simulink model "auv_v3_closed_loop"  (R2024b)
settings: Solver=ode4  StartTime=0.0  StopTime=200  FixedStep=0.02  RelTol=1e-3
model workspace (MAT data in the model file):
  CaseIndex = 1
  ControllerMode = 2
settings Model: Creator=HakugyoMyon  LastModifiedBy=HakugyoMyon
settings DataIOCC: SaveOutput=off

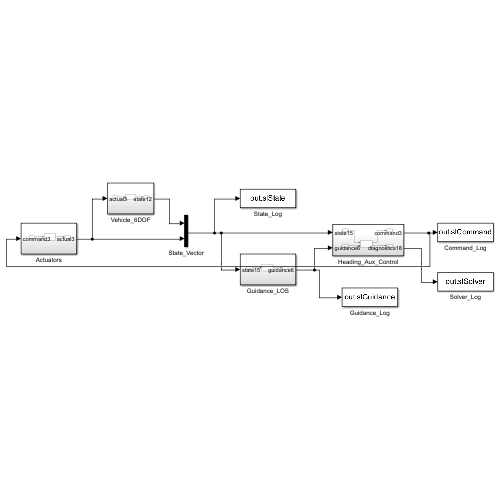
[thumbnail: Simulink's stored preview of the top-level diagram]
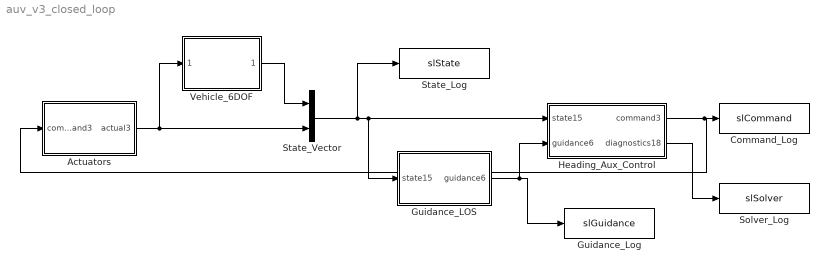
== system auv_v3_closed_loop ==
  Actuators : Subsystem
  Command_Log : ToWorkspace  VariableName=slCommand  SaveFormat=Timeseries  SampleTime=0.1
  Guidance_LOS : Subsystem
  Guidance_Log : ToWorkspace  VariableName=slGuidance  SaveFormat=Timeseries  SampleTime=0.1
  Heading_Aux_Control : Subsystem
  Solver_Log : ToWorkspace  VariableName=slSolver  SaveFormat=Timeseries  SampleTime=0.1
  State_Log : ToWorkspace  VariableName=slState  SaveFormat=Timeseries  SampleTime=0.1
  State_Vector : Mux  Inputs=2
  Vehicle_6DOF : Subsystem
  wires:
  Heading_Aux_Control/2(diagnostics18) -> Solver_Log/1
  Heading_Aux_Control/1(command3) -> Command_Log/1, Actuators/1(command3)
  Guidance_LOS/1(guidance6) -> Guidance_Log/1, Heading_Aux_Control/2(guidance6)
  State_Vector/1 -> Guidance_LOS/1(state15), Heading_Aux_Control/1(state15), State_Log/1
  Actuators/1(actual3) -> State_Vector/2, Vehicle_6DOF/1(actual3)
  Vehicle_6DOF/1(state12) -> State_Vector/1

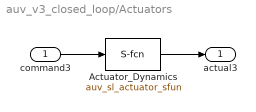
== system auv_v3_closed_loop/Actuators ==
  command3 : Inport
  Actuator_Dynamics : M-S-Function  FunctionName=auv_sl_actuator_sfun  Parameters=CaseIndex
  actual3 : Outport
  wires:
  Actuator_Dynamics/1 -> actual3/1
  command3/1 -> Actuator_Dynamics/1

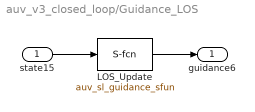
== system auv_v3_closed_loop/Guidance_LOS ==
  state15 : Inport
  LOS_Update : M-S-Function  FunctionName=auv_sl_guidance_sfun  Parameters=CaseIndex
  guidance6 : Outport
  wires:
  LOS_Update/1 -> guidance6/1
  state15/1 -> LOS_Update/1

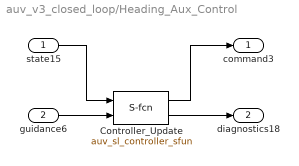
== system auv_v3_closed_loop/Heading_Aux_Control ==
  state15 : Inport
  guidance6 : Inport  Port=2
  Controller_Update : M-S-Function  FunctionName=auv_sl_controller_sfun  Parameters=CaseIndex,ControllerMode
  command3 : Outport
  diagnostics18 : Outport  Port=2
  wires:
  Controller_Update/2 -> diagnostics18/1
  Controller_Update/1 -> command3/1
  guidance6/1 -> Controller_Update/2
  state15/1 -> Controller_Update/1

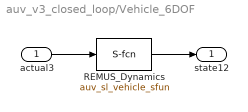
== system auv_v3_closed_loop/Vehicle_6DOF ==
  actual3 : Inport
  REMUS_Dynamics : M-S-Function  FunctionName=auv_sl_vehicle_sfun  Parameters=CaseIndex
  state12 : Outport
  wires:
  REMUS_Dynamics/1 -> state12/1
  actual3/1 -> REMUS_Dynamics/1
